simulink model "second_order"  (R2025b)
settings: Solver=FixedStepAuto  StartTime=0.0  StopTime=10  FixedStep=0.001  RelTol=1e-6
InitFcn:
  | % % Tunable knob
  | % T_set = 200;
  | % s_CL = -6/T_set;
  | % % Kp = s_CL^2;
  | % % Kd = -2*s_CL;
  | %
  | % % Kp = 0.001064;
  | % % Kd = 0.063514;
  | %
  | % % Kp = 0.000537;
  | % % Kd = 0.038196;
  | %
  | % % Kp = 0.00045;
  | % % Kd = 0.040196;
  | %
  | %             Kp = 0.0003;
  | %             Kd = 0.09;
  | %
  | % Kob = 10;
  | %
  | % %             K = 164.458741/50*1;
  | % % tau1 = 160.525043;
  | % % tau2 = 835.747525;
  | % %             L_comp = 13.297226;
  | % %             L_sys  = 13.297226;
  | % K = 1.467057642011806*2;
  | % K0 = 1.467057642011806*2;
  | % tau1 = 5.108331033027039e+02;
  | % tau2 = 35.728915073943433;
  | % L_comp = 15.024369999999999;
  | % L_sys = 15.024369999999999;
  | % % K = 1.455368;
  | % % K0 = 1.455368;
  | % % tau1 = 18.226428;
  | % % tau2 = 538.493088;
  | % % L_comp = 33.344271;
  | % % L_sys = 33.344271;
  | % t1 = tau1*tau2;
  | % b0 = K0/t1;
  | %
  | % % Derived quantities
  | % s_ESO = Kob*s_CL;
  | % l1 = -3*s_ESO;
  | % l2 = 3*s_ESO^2;
  | % l3 = -s_ESO^3;
  | %
  | % A = [-l1  1  0;
  | %      -l2  0  1
  | %      -l3  0  0];
  | %
  | % B = [0   l1
  | %      b0  l2;
  | %      0   l3];
  | %
  | % % discrete equivalent
  | % Ts = 0.005;
  | % Ad = [1  Ts  Ts^2/2
  | %       0   1      Ts
  | %       0   0       1];
  | % Bd = [b0*Ts^2/2; b0*Ts; 0];
  | % z_ESO = exp(s_ESO*Ts);
  | % dl1 = 1-z_ESO^3;
  | % dl2 = 3/(2*Ts) * (1-z_ESO)^2*(1+z_ESO);
  | % dl3 = 1/Ts^2 * (1-z_ESO)^3;
  | % Cd = [1 0 0]; Ld = [dl1;dl2;dl3];
  | % Aeso = Ad - Ld*Cd*Ad;
  | % Beso = Bd - Ld*Cd*Bd;
  | % delay_comp = round(L_comp*200);
  | % delay_sys  = round(L_sys*200);
  | % K1 = Kp; K2 = Kd;
  | 
  | 
  | 
  | % Tunable knob
  | T_set = 200;
  | s_CL = -6/T_set;
  | % Kp = s_CL^2;
  | % Kd = -2*s_CL;
  | Kp = 0.00055;
  | Kd = 0.06;
  | 
  | Kob = 2;
  | 
  | K = 1.6937;
  | K0 = 1.6937 ;
  | tau1 = 792.76;
  | tau2 = 56.103;
  | L_comp = 29.97;
  | L_sys = 29.97;
  | t1 = tau1*tau2;
  | b0 = K0/t1;
  | 
  | % Derived quantities
  | s_ESO = Kob*s_CL;
  | l1 = -3*s_ESO;
  | l2 = 3*s_ESO^2;
  | l3 = -s_ESO^3;
  | 
  | A = [-l1  1  0;
  |      -l2  0  1
  |      -l3  0  0];
  | 
  | B = [0   l1
  |      b0  l2;
  |      0   l3];
  | 
  | % discrete equivalent
  | Ts = 0.005;
  | Ad = [1  Ts  Ts^2/2
  |       0   1      Ts
  |       0   0       1];
  | Bd = [b0*Ts^2/2; b0*Ts; 0];
  | z_ESO = exp(s_ESO*Ts);
  | dl1 = 1-z_ESO^3;
  | dl2 = 3/(2*Ts) * (1-z_ESO)^2*(1+z_ESO);
  | dl3 = 1/Ts^2 * (1-z_ESO)^3;
  | Cd = [1 0 0]; Ld = [dl1;dl2;dl3];
  | Aeso = Ad - Ld*Cd*Ad;
  | Beso = Bd - Ld*Cd*Bd;
  | delay_comp = round(L_comp*200);
  | delay_sys  = round(L_sys*200);
  | K1 = Kp; K2 = Kd;
libraries: simulink x4
settings Model: Creator=SARIR  LastModifiedBy=MG8102
settings RTWCC: GPUComputeCapability=3.5

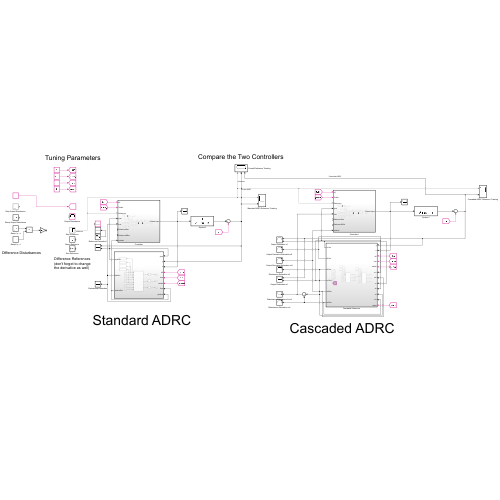
[thumbnail: Simulink's stored preview of the top-level diagram]
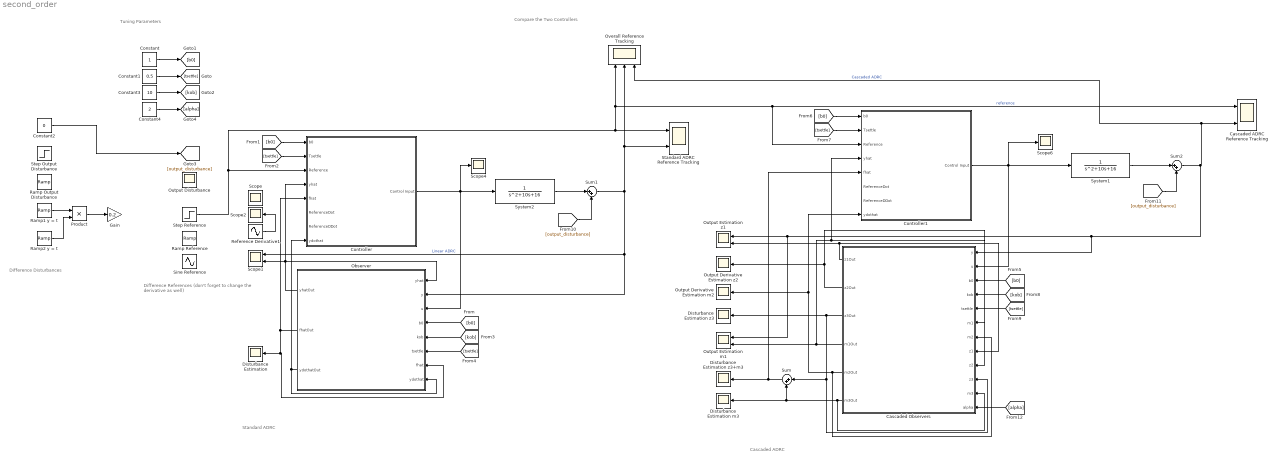
== system second_order ==
  note: Cascaded ADRC
  note: Difference References
      | (don't forget to change the derivative as well)
  note: Standard ADRC
  note: Tuning Parameters
  note: Difference Disturbances
  note: Compare the Two Controllers
  Cascaded ADRC Reference Tracking : Scope  NumInputPorts=2
      settings: ActiveDisplayYMinimum=-0.12499999999999997  ActiveDisplayYMaximum=1.125  DataLoggingVariableName=ScopeData11
  Cascaded Observers : Subsystem
  Constant : Constant
  Constant1 : Constant  Value=0.5
  Constant2 : Constant  Value=0
  Constant3 : Constant  Value=10
  Constant4 : Constant  Value=2
  Controller : Subsystem
  Controller1 : Subsystem
  Disturbance Estimation : Scope
      settings: ActiveDisplayYMinimum=-1  ActiveDisplayYMaximum=1  DataLoggingVariableName=ScopeData2
  Disturbance Estimation m3 : Scope
      settings: ActiveDisplayYMinimum=-0.17051590917545686  ActiveDisplayYMaximum=0.28464522778338275  DataLoggingVariableName=ScopeData14
  Disturbance Estimation z3 : Scope
      settings: ActiveDisplayYMinimum=-14.202723242399511  ActiveDisplayYMaximum=4.0163647793875974  DataLoggingVariableName=ScopeData3
  Disturbance Estimation z3+m3 : Scope
      settings: ActiveDisplayYMinimum=-14.368421578921289  ActiveDisplayYMaximum=4.2576518564936743  DataLoggingVariableName=ScopeData15
  Gain : Gain  Gain=0.2
  Observer : Subsystem
  Output Derivative Estimation m2 : Scope
      settings: ActiveDisplayYMinimum=-14.202723242399511  ActiveDisplayYMaximum=4.0163647793875974  DataLoggingVariableName=ScopeData26
  Output Derivative Estimation z2 : Scope
      settings: ActiveDisplayYMinimum=-14.202723242399511  ActiveDisplayYMaximum=4.0163647793875974  DataLoggingVariableName=ScopeData25
  Output Disturbance : Scope
      settings: ActiveDisplayYMinimum=-1  ActiveDisplayYMaximum=1  DataLoggingVariableName=ScopeData17
  Output Estimation m1 : Scope  NumInputPorts=2
      settings: ActiveDisplayYMinimum=-0.11700544897399281  ActiveDisplayYMaximum=1.0530490407659356  DataLoggingVariableName=ScopeData16
  Output Estimation z1 : Scope  NumInputPorts=2
      settings: ActiveDisplayYMinimum=-0.11700544897399281  ActiveDisplayYMaximum=1.0530490407659356  DataLoggingVariableName=ScopeData8
  Overall Reference Tracking : Scope  NumInputPorts=3
      settings: ActiveDisplayYMinimum=-0.12531748060479711  ActiveDisplayYMaximum=1.1278573254431743  DataLoggingVariableName=ScopeData18
  Product : Product
  Ramp Output Disturbance : simulink/Sources/Ramp  slope=.5  start=5  InitialOutput=0
  Ramp Reference : simulink/Sources/Ramp  slope=1  start=2  InitialOutput=0
  Ramp1 y = t : simulink/Sources/Ramp  slope=1  start=5  InitialOutput=0
  Ramp2 y = t : simulink/Sources/Ramp  slope=1  start=5  InitialOutput=0
  Reference Derivative1 : Sin  Amplitude=2  Frequency=2  Phase=pi/2  SampleTime=0
  Scope{,2,4,6} (4 alike) : Scope
      Scope settings: ActiveDisplayYMinimum=-1  ActiveDisplayYMaximum=1  DataLoggingVariableName=ScopeData19
      Scope2 settings: ActiveDisplayYMinimum=-1  ActiveDisplayYMaximum=1  DataLoggingVariableName=ScopeData20
      Scope4 settings: ActiveDisplayYMinimum=-2.1349074056818003  ActiveDisplayYMaximum=29.734332855269823  DataLoggingVariableName=ScopeData13
      Scope6 settings: ActiveDisplayYMinimum=-2.1349074056818003  ActiveDisplayYMaximum=29.734332855269823  DataLoggingVariableName=ScopeData12
  Scope1 : Scope  NumInputPorts=2
      settings: ActiveDisplayYMinimum=-0.12500000000000422  ActiveDisplayYMaximum=1.1250000000000382
  Sine Reference : Sin  Frequency=2  SampleTime=0
  Standard ADRC Reference Tracking : Scope  NumInputPorts=2
      settings: ActiveDisplayYMinimum=-0.12499999999999997  ActiveDisplayYMaximum=1.125
  Step Output Disturbance : Step  Time=5  After=0.5  SampleTime=0
  Step Reference : Step  Time=2  SampleTime=0
  Sum : Sum  Inputs=|++
  Sum1 : Sum  Inputs=|++
  Sum2 : Sum  Inputs=|++
  System1 : TransferFcn  Denominator=[1 10 16]
  System2 : TransferFcn  Denominator=[1 10 16]
  wires:
  Observer/2(fhatOut) -> Controller/5(fhat), Observer/7(fhat), Disturbance Estimation/1
  [b0] -> Observer/4(b0)
  Constant/1 -> [b0]
  [b0] -> Controller/1(b0)
  [tsettle] -> Controller/2(Tsettle)
  [tsettle] -> Observer/6(tsettle)
  Constant1/1 -> [tsettle]
  Constant3/1 -> [kob]
  [kob] -> Observer/5(kob)
  Observer/1(yhatOut) -> Observer/1(yhat), Controller/4(yhat), Scope1/2
  Controller/1(Control Input) -> Scope4/1, Observer/3(u), System2/1
  [tsettle] -> Controller1/2(Tsettle)
  [kob] -> Cascaded Observers/4(kob)
  [tsettle] -> Cascaded Observers/5(tsettle)
  Controller1/1(Control Input) -> Scope6/1, System1/1, Cascaded Observers/2(u)
  [b0] -> Controller1/1(b0)
  [b0] -> Cascaded Observers/3(b0)
  Sum/1 -> Controller1/5(fhat), Disturbance Estimation z3+m3/1
  Cascaded Observers/2(z2Out) -> Cascaded Observers/9(z2), Output Derivative Estimation z2/1
  System2/1 -> Sum1/1
  [output_disturbance] -> Sum1/2
  Sum1/1 -> Observer/2(y), Scope1/1, Standard ADRC Reference Tracking/2, Overall Reference Tracking/2  "Linear ADRC"
  Sum2/1 -> Cascaded ADRC Reference Tracking/2, Overall Reference Tracking/3, Output Estimation m1/1, Output Estimation z1/1, Cascaded Observers/1(y)  "Cascaded ADRC"
  System1/1 -> Sum2/1
  [output_disturbance] -> Sum2/2
  Ramp1 y = t/1 -> Product/1
  Ramp2 y = t/1 -> Product/2
  Product/1 -> Gain/1
  Reference Derivative1/1 -> Scope2/1
  Step Reference/1 -> Overall Reference Tracking/1, Controller1/3(Reference), Cascaded ADRC Reference Tracking/1, Standard ADRC Reference Tracking/1, Controller/3(Reference)  "reference"
  Observer/3(ydothatOut) -> Observer/8(ydothat), Controller/8(ydothat)
  Cascaded Observers/4(m1Out) -> Controller1/4(yhat), Cascaded Observers/6(m1), Output Estimation m1/2
  Cascaded Observers/3(z3Out) -> Sum/1, Cascaded Observers/10(z3), Disturbance Estimation z3/1
  Cascaded Observers/6(m3Out) -> Sum/2, Disturbance Estimation m3/1, Cascaded Observers/11(m3)
  Cascaded Observers/1(z1Out) -> Output Estimation z1/2, Cascaded Observers/8(z1)
  Cascaded Observers/5(m2Out) -> Cascaded Observers/7(m2), Controller1/8(ydothat), Output Derivative Estimation m2/1
  Constant2/1 -> [output_disturbance]
  Constant4/1 -> [alpha]
  [alpha] -> Cascaded Observers/12(alpha)

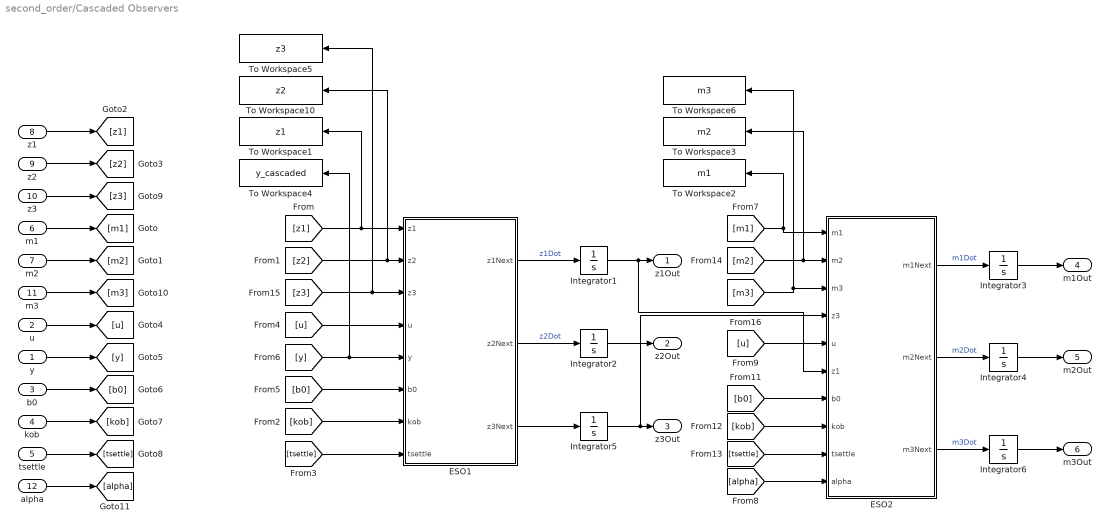
== system second_order/Cascaded Observers ==
  y : Inport
  u : Inport  Port=2
  b0 : Inport  Port=3
  kob : Inport  Port=4
  tsettle : Inport  Port=5
  m1 : Inport  Port=6
  m2 : Inport  Port=7
  z1 : Inport  Port=8
  z2 : Inport  Port=9
  z3 : Inport  Port=10
  m3 : Inport  Port=11
  alpha : Inport  Port=12
  ESO1 : MATLAB Function  TreatAsAtomicUnit=on
  ESO2 : MATLAB Function  TreatAsAtomicUnit=on
  Integrator{1..6} (6 alike) : Integrator
  To Workspace1 : ToWorkspace  VariableName=z1  SaveFormat=Timeseries  SampleTime=-1
  To Workspace10 : ToWorkspace  VariableName=z2  SaveFormat=Timeseries  SampleTime=-1
  To Workspace2 : ToWorkspace  VariableName=m1  SaveFormat=Timeseries  SampleTime=-1
  To Workspace3 : ToWorkspace  VariableName=m2  SaveFormat=Timeseries  SampleTime=-1
  To Workspace4 : ToWorkspace  VariableName=y_cascaded  SaveFormat=Timeseries  SampleTime=-1
  To Workspace5 : ToWorkspace  VariableName=z3  SaveFormat=Timeseries  SampleTime=-1
  To Workspace6 : ToWorkspace  VariableName=m3  SaveFormat=Timeseries  SampleTime=-1
  z1Out : Outport
  z2Out : Outport  Port=2
  z3Out : Outport  Port=3
  m1Out : Outport  Port=4
  m2Out : Outport  Port=5
  m3Out : Outport  Port=6
  wires:
  [b0] -> ESO1/6(b0)
  ESO1/1(z1Next) -> Integrator1/1  "z1Dot"
  [kob] -> ESO1/7(kob)
  [z1] -> To Workspace1/1, ESO1/1(z1)
  [tsettle] -> ESO1/8(tsettle)
  [u] -> ESO1/4(u)
  [y] -> To Workspace4/1, ESO1/5(y)
  ESO1/2(z2Next) -> Integrator2/1  "z2Dot"
  [z2] -> To Workspace10/1, ESO1/2(z2)
  ESO2/2(m2Next) -> Integrator4/1  "m2Dot"
  ESO2/1(m1Next) -> Integrator3/1  "m1Dot"
  Integrator2/1 -> z2Out/1
  Integrator4/1 -> m2Out/1
  Integrator3/1 -> m1Out/1
  m1/1 -> [m1]
  m2/1 -> [m2]
  z1/1 -> [z1]
  z2/1 -> [z2]
  tsettle/1 -> [tsettle]
  kob/1 -> [kob]
  b0/1 -> [b0]
  y/1 -> [y]
  u/1 -> [u]
  [m2] -> To Workspace3/1, ESO2/2(m2)
  [m1] -> To Workspace2/1, ESO2/1(m1)
  [u] -> ESO2/5(u)
  Integrator1/1 -> ESO2/6(z1), z1Out/1
  [b0] -> ESO2/7(b0)
  [kob] -> ESO2/8(kob)
  [tsettle] -> ESO2/9(tsettle)
  ESO1/3(z3Next) -> Integrator5/1
  z3/1 -> [z3]
  m3/1 -> [m3]
  [z3] -> To Workspace5/1, ESO1/3(z3)
  Integrator5/1 -> ESO2/4(z3), z3Out/1
  [m3] -> ESO2/3(m3), To Workspace6/1
  ESO2/3(m3Next) -> Integrator6/1  "m3Dot"
  Integrator6/1 -> m3Out/1
  alpha/1 -> [alpha]
  [alpha] -> ESO2/10(alpha)

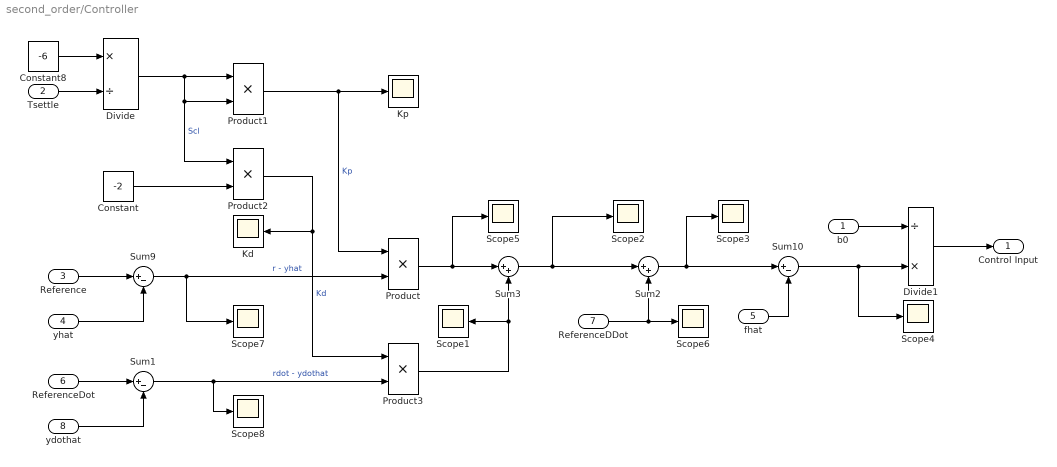
== system second_order/Controller ==
  b0 : Inport
  Tsettle : Inport  Port=2
  Reference : Inport  Port=3
  yhat : Inport  Port=4
  fhat : Inport  Port=5
  ReferenceDot : Inport  Port=6
  ReferenceDDot : Inport  Port=7
  ydothat : Inport  Port=8
  Constant : Constant  Value=-2
  Constant8 : Constant  Value=-6
  Divide : Product  Inputs=*/
  Divide1 : Product  Inputs=/*
  Kd : Scope
      settings: ActiveDisplayYMinimum=-1  ActiveDisplayYMaximum=1  DataLoggingVariableName=ScopeData23
  Kp : Scope
      settings: ActiveDisplayYMinimum=-1  ActiveDisplayYMaximum=1  DataLoggingVariableName=ScopeData4
  Product{,1..3} (4 alike) : Product
  Scope{1..8} (8 alike) : Scope
      Scope1 settings: ActiveDisplayYMinimum=-1  ActiveDisplayYMaximum=1  DataLoggingVariableName=ScopeData24
      Scope2 settings: ActiveDisplayYMinimum=-1  ActiveDisplayYMaximum=1  DataLoggingVariableName=ScopeData5
      Scope3 settings: ActiveDisplayYMinimum=-1  ActiveDisplayYMaximum=1  DataLoggingVariableName=ScopeData6
      Scope4 settings: ActiveDisplayYMinimum=-1  ActiveDisplayYMaximum=1  DataLoggingVariableName=ScopeData7
      Scope5 settings: ActiveDisplayYMinimum=-653.59068328826925  ActiveDisplayYMaximum=704.60718213499831  DataLoggingVariableName=ScopeData21
      Scope6 settings: ActiveDisplayYMinimum=-1  ActiveDisplayYMaximum=1  DataLoggingVariableName=ScopeData9
      Scope7 settings: ActiveDisplayYMinimum=-0.12499999999999997  ActiveDisplayYMaximum=1.125  DataLoggingVariableName=ScopeData10
      Scope8 settings: ActiveDisplayYMinimum=-1510.7201089209848  ActiveDisplayYMaximum=1425.0890988962974  DataLoggingVariableName=ScopeData22
  Sum1 : Sum  Inputs=|+-
  Sum10 : Sum  Inputs=|+-
  Sum2 : Sum  Inputs=|++
  Sum3 : Sum  Inputs=|++
  Sum9 : Sum  Inputs=|+-
  Control Input : Outport
  wires:
  Divide1/1 -> Control Input/1
  Constant8/1 -> Divide/1
  Sum9/1 -> Scope7/1, Product/2  "r - yhat"
  yhat/1 -> Sum9/2
  Tsettle/1 -> Divide/2
  Sum10/1 -> Scope4/1, Divide1/2
  Reference/1 -> Sum9/1
  b0/1 -> Divide1/1
  fhat/1 -> Sum10/2
  Sum2/1 -> Scope3/1, Sum10/1
  Divide/1 -> Product1/2, Product2/1, Product1/1  "Scl"
  Constant/1 -> Product2/2
  Product1/1 -> Kp/1, Product/1  "Kp"
  ReferenceDDot/1 -> Sum2/2, Scope6/1
  ReferenceDot/1 -> Sum1/1
  ydothat/1 -> Sum1/2
  Product2/1 -> Kd/1, Product3/1  "Kd"
  Sum1/1 -> Scope8/1, Product3/2  "rdot - ydothat"
  Product/1 -> Scope5/1, Sum3/1
  Product3/1 -> Scope1/1, Sum3/2
  Sum3/1 -> Scope2/1, Sum2/1

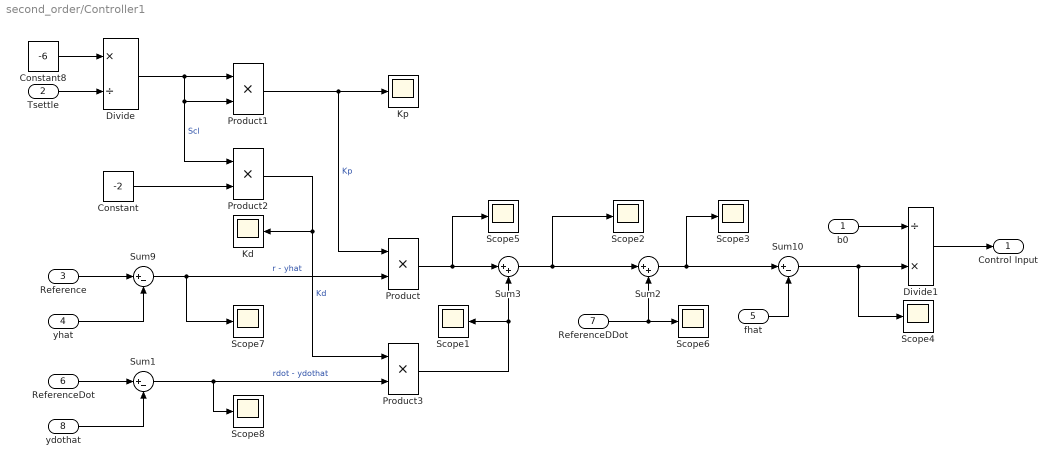
== system second_order/Controller1 ==
  b0 : Inport
  Tsettle : Inport  Port=2
  Reference : Inport  Port=3
  yhat : Inport  Port=4
  fhat : Inport  Port=5
  ReferenceDot : Inport  Port=6
  ReferenceDDot : Inport  Port=7
  ydothat : Inport  Port=8
  Constant : Constant  Value=-2
  Constant8 : Constant  Value=-6
  Divide : Product  Inputs=*/
  Divide1 : Product  Inputs=/*
  Kd : Scope
      settings: ActiveDisplayYMinimum=-1  ActiveDisplayYMaximum=1  DataLoggingVariableName=ScopeData23
  Kp : Scope
      settings: ActiveDisplayYMinimum=-1  ActiveDisplayYMaximum=1  DataLoggingVariableName=ScopeData4
  Product{,1..3} (4 alike) : Product
  Scope{1..8} (8 alike) : Scope
      Scope1 settings: ActiveDisplayYMinimum=0.26  ActiveDisplayYMaximum=0.46  DataLoggingVariableName=ScopeData24
      Scope2 settings: ActiveDisplayYMinimum=-0.04519  ActiveDisplayYMaximum=0.40502  DataLoggingVariableName=ScopeData5
      Scope3 settings: ActiveDisplayYMinimum=-0.1955  ActiveDisplayYMaximum=1.75506  DataLoggingVariableName=ScopeData6
      Scope4 settings: ActiveDisplayYMinimum=-0.195  ActiveDisplayYMaximum=1.755  DataLoggingVariableName=ScopeData7
      Scope5 settings: ActiveDisplayYMinimum=0.26  ActiveDisplayYMaximum=0.46  DataLoggingVariableName=ScopeData21
      Scope6 settings: ActiveDisplayYMinimum=-0.40718  ActiveDisplayYMaximum=1.15635  DataLoggingVariableName=ScopeData9
      Scope7 settings: ActiveDisplayYMinimum=-0.12554  ActiveDisplayYMaximum=1.12506  DataLoggingVariableName=ScopeData10
      Scope8 settings: ActiveDisplayYMinimum=0.26  ActiveDisplayYMaximum=0.46  DataLoggingVariableName=ScopeData22
  Sum1 : Sum  Inputs=|+-
  Sum10 : Sum  Inputs=|+-
  Sum2 : Sum  Inputs=|++
  Sum3 : Sum  Inputs=|++
  Sum9 : Sum  Inputs=|+-
  Control Input : Outport
  wires:
  Divide1/1 -> Control Input/1
  Constant8/1 -> Divide/1
  Sum9/1 -> Scope7/1, Product/2  "r - yhat"
  yhat/1 -> Sum9/2
  Tsettle/1 -> Divide/2
  Sum10/1 -> Scope4/1, Divide1/2
  Reference/1 -> Sum9/1
  b0/1 -> Divide1/1
  fhat/1 -> Sum10/2
  Sum2/1 -> Scope3/1, Sum10/1
  Divide/1 -> Product1/2, Product2/1, Product1/1  "Scl"
  Constant/1 -> Product2/2
  Product1/1 -> Kp/1, Product/1  "Kp"
  ReferenceDDot/1 -> Sum2/2, Scope6/1
  ReferenceDot/1 -> Sum1/1
  ydothat/1 -> Sum1/2
  Product2/1 -> Kd/1, Product3/1  "Kd"
  Sum1/1 -> Scope8/1, Product3/2  "rdot - ydothat"
  Product/1 -> Scope5/1, Sum3/1
  Product3/1 -> Scope1/1, Sum3/2
  Sum3/1 -> Scope2/1, Sum2/1

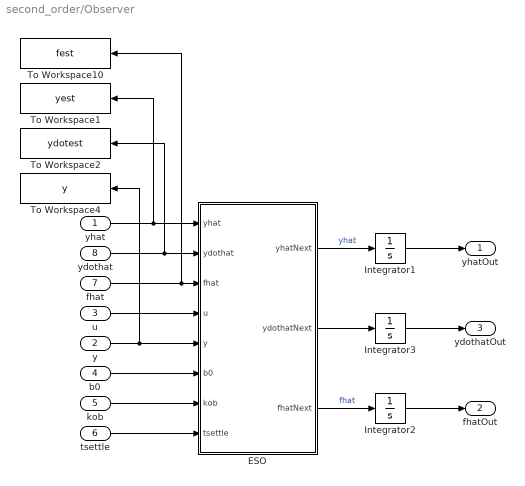
== system second_order/Observer ==
  yhat : Inport
  y : Inport  Port=2
  u : Inport  Port=3
  b0 : Inport  Port=4
  kob : Inport  Port=5
  tsettle : Inport  Port=6
  fhat : Inport  Port=7
  ydothat : Inport  Port=8
  ESO : MATLAB Function  TreatAsAtomicUnit=on
  Integrator1 : Integrator
  Integrator2 : Integrator
  Integrator3 : Integrator
  To Workspace1 : ToWorkspace  VariableName=yest  SaveFormat=Timeseries  SampleTime=-1
  To Workspace10 : ToWorkspace  VariableName=fest  SaveFormat=Timeseries  SampleTime=-1
  To Workspace2 : ToWorkspace  VariableName=ydotest  SaveFormat=Timeseries  SampleTime=-1
  To Workspace4 : ToWorkspace  VariableName=y  SaveFormat=Timeseries  SampleTime=-1
  yhatOut : Outport
  fhatOut : Outport  Port=2
  ydothatOut : Outport  Port=3
  wires:
  b0/1 -> ESO/6(b0)
  ESO/1(yhatNext) -> Integrator1/1  "yhat"
  kob/1 -> ESO/7(kob)
  yhat/1 -> To Workspace1/1, ESO/1(yhat)
  tsettle/1 -> ESO/8(tsettle)
  u/1 -> ESO/4(u)
  y/1 -> To Workspace4/1, ESO/5(y)
  ESO/3(fhatNext) -> Integrator2/1  "fhat"
  fhat/1 -> To Workspace10/1, ESO/3(fhat)
  Integrator1/1 -> yhatOut/1
  Integrator2/1 -> fhatOut/1
  ydothat/1 -> To Workspace2/1, ESO/2(ydothat)
  ESO/2(ydothatNext) -> Integrator3/1
  Integrator3/1 -> ydothatOut/1

== matlab function second_order/Cascaded Observers/ESO1 ==
  data: z1 input; z2 input; z3 input; u input; z1Next output; y input; b0 input; kob input; tsettle input; z2Next output; z3Next output
function [z1Next, z2Next, z3Next] = fcn(z1, z2, z3, u, y, b0, kob, tsettle)
    Scl = -6/tsettle;
    Seso = kob * Scl;

    l1 = -3 * Seso;
    l2 = 3*(Seso^2);
    l3 = -(Seso^3);
    
    A = [0, 1, 0; 0, 0, 1; 0, 0, 0]; 
    B = [0; b0; 0];
    C = [1, 0, 0];
    D = 0;
    L = [l1; l2; l3];

    zPrev = [z1; z2; z3]; 
    zNext = A * zPrev + B * u + L * (y - C*zPrev);
     
    z1Next = zNext(1);
    z2Next = zNext(2);
    z3Next = zNext(3);

== matlab function second_order/Observer/ESO ==
  data: yhat input; ydothat input; fhat input; u input; yhatNext output; ydothatNext output; y input; b0 input; kob input; tsettle input; fhatNext output
function [yhatNext, ydothatNext, fhatNext] = fcn(yhat, ydothat, fhat, u, y, b0, kob, tsettle)
    Scl = -6/tsettle;
    Seso = kob * Scl;

    l1 = -3 * Seso;
    l2 = 3*(Seso^2);
    l3 = -(Seso^3);
    
    A = [0, 1, 0; 0, 0, 1; 0, 0, 0]; 
    B = [0; b0; 0];
    C = [1, 0, 0];
    D = 0;
    L = [l1; l2; l3];

    xPrev = [yhat; ydothat; fhat]; 
    xNext = A * xPrev + B * u + L * (y - C*xPrev);
     
    yhatNext = xNext(1);
    ydothatNext = xNext(2);
    fhatNext = xNext(3);

== matlab function second_order/Cascaded Observers/ESO2 ==
  data: m1 input; m2 input; m3 input; z3 input; u input; m1Next output; z1 input; b0 input; kob input; tsettle input; m2Next output; m3Next output; alpha input
function [m1Next, m2Next, m3Next] = fcn(m1, m2, m3, z3, u, z1, b0, kob, tsettle, alpha)
    Scl = -6/tsettle;
    Seso = kob * Scl * alpha;

    l1 = -3 * Seso;
    l2 = 3*(Seso^2);
    l3 = -(Seso^3);
    
    A = [0, 1, 0; 0, 0, 1; 0, 0, 0]; 
    B = [0; b0; 0];
    C = [1, 0, 0];
    D = 0;
    L = [l1; l2; l3];

    mPrev = [m1; m2; m3]; 
    mNext = A * mPrev + B * u + L * (z1 - C*mPrev) + [0; z3; 0];
     
    m1Next = mNext(1);
    m2Next = mNext(2);
    m3Next = mNext(3);
